simulink model "WSCC01"  (R2024b)
settings: Solver=ode23tb  StartTime=0.0  StopTime=110  MaxStep=1/60  RelTol=1e-4  AbsTol=1e-3  EnableMultiTasking=on
InitFcn:
  | PSSMODEL=1;
  | MB=[1   0.2 30   1.25 40    12 160];
  | 
  | k=[8.3222    2.6014   19.0811    1.9818    3.6841   19.1783  240.6785    2.5684    4.3666   58.7391 7.6960   47.7975    8.7139  296.2463    2.7543    6.5051   47.7755    0.4780   35.4950   18.1866 94.2186]
  | k1=k(1);
  | k2=k(2);
  | k3=k(3);
  | k4=k(4);
  | k5=k(5);
  | k6=k(6);
  | k7=k(7);
  | k8=k(8);
  | k9=k(9);
  | k10=k(10);
  | k11=k(11);
  | k12=k(12);
  | k13=k(13);
  | k14=k(14);
  | k15=k(15);
  | k16=k(16);
  | k17=k(17);
  | k18=k(18);
  | k19=k(19);
  | k20=k(20);
  | k21=k(21);
libraries: spsThreePhaseVIMeasurementLib x12, spsLoadFlowBusLib x9, spsThreePhasePISectionLineLib x6, spsThreePhaseTransformerTwoWindingsLib x3, spsSynchronousMachinepuStandardLib x3, spsExcitationSystemLib x3, spsMultiBandPowerSystemStabilizerLib x3, spsSteamTurbineandGovernorLib x3, spsThreePhaseParallelRLCLoadLib x3, spsThreePhaseDynamicLoadLib x1, spspowerguiLib x1
settings Model: Creator=jp536285  LastModifiedBy=Raju
settings SolverCC: AutoScaleAbsTol=off  AlgebraicLoopSolver=TrustRegion
settings OptimizationCC: LifeSpan=inf
settings DebuggingCC: UnderspecifiedInitializationDetection=Classic  MergeDetectMultiDrivingBlocksExec=none  SolverPrmCheckMsg=warning  StateNameClashWarn=warning  SFUnexpectedBacktrackingDiag=warning  SFNoUnconditionalDefaultTransitionDiag=warning  ArithmeticOperatorsInVariantConditions=warning
settings HardwareCC: ProdBitPerPointer=32  ProdBitPerSizeT=32  ProdBitPerPtrDiffT=32  ProdLargestAtomicFloat=None  ProdIntDivRoundTo=Undefined  ProdEndianess=Unspecified  ProdWordSize=32  ProdHWDeviceType=32-bit Generic
settings ModelReferenceCC: EnableRefExpFcnMdlSchedulingChecks=on  PropagateSignalLabelsOutOfModel=off
settings SFSimCC: SimUseLocalCustomCode=off  CustomCodeUndefinedFunction=UseInterfaceOnly
settings RTWCC: RTWUseLocalCustomCode=off  GPUComputeCapability=3.5
settings CodeAppCC: StateflowObjectComments=on
settings GRTTargetCC: TargetLangStandard=C89/C90 (ANSI)
settings ConfigComp: CovMetricSettings=dw  CovSaveCumulativeToWorkspaceVar=on  CovSaveSingleToWorkspaceVar=on  CovExternalEMLEnable=off
settings SimscapeCC: SimscapeNormalizeSystem=off

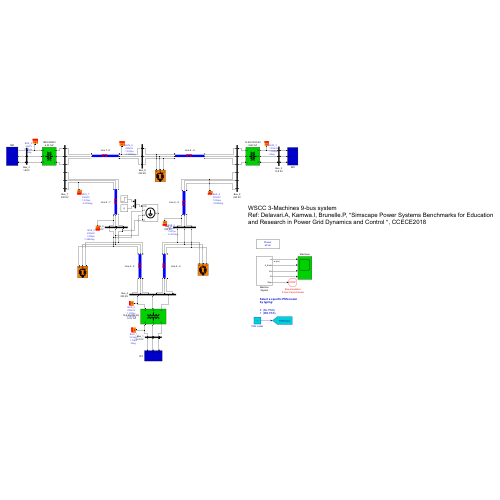
[thumbnail: Simulink's stored preview of the top-level diagram]
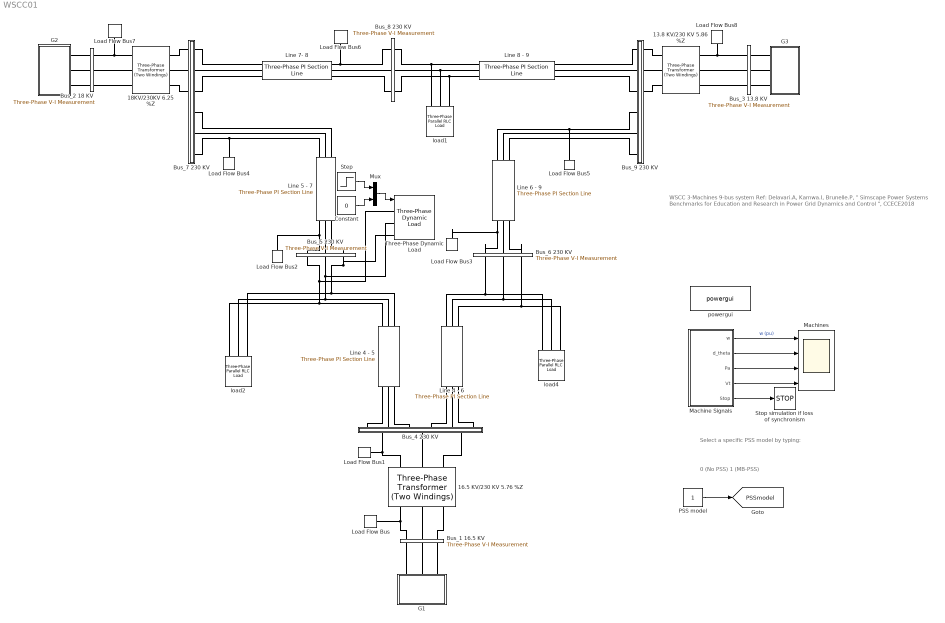
== system WSCC01 ==
  note: WSCC 3-Machines 9-bus system
      | Ref: Delavari.A, Kamwa.I, Brunelle.P, " Simscape Power Systems Benchmarks for Education
      | and Research in Power Grid Dynamics and Control ", CCECE2018
  note: Select a specific PSS model
      | by typing:
  note: 0  (No PSS)
      | 1  (MB-PSS)
  " Line 4 - 6" : spsThreePhasePISectionLineLib/Three-Phase PI Section Line  LConnTagsString=a|b|c  RConnTagsString=A|B|C  Length=100  Frequency=60  Resistances=[ 0.08993 0.224825]  Inductances="[ 1.29e-3  3.22e-3]"  Capacitances="[ 9.5e-9  6.5e-9 ]"  mask(Three-Phase PI Section Line){}
      mask Display:
      | % This is a new mask on top of the base mask.
      | % Use "View base mask" link below to see the base mask.
      | patch([0.0 0.0 1 1 0.0 0.0 ],[0.4 0.7 0.7 0.4 0.4 0.7],[0 0 1]);
      | patch([0.4 0.4 0.42 0.42],[0.4 0.75 0.75 0.4],[1 0 0]);
      | patch([0.38 0.38 0.57 0.57],[0.7 0.75 0.75 0.7],[1 0 0]);
      | patch([0.53 0.53 0.55 0.55],[0.4 0.75 0.75 0.4],[1 0 0]);
  " Line 6 - 9" : spsThreePhasePISectionLineLib/Three-Phase PI Section Line  LConnTagsString=a|b|c  RConnTagsString=A|B|C  Length=100  Frequency=60  Resistances=[ 0.20631 0.5157]  Inductances="[ 2.38e-3  6.09e-3]"  Capacitances=[17.95e-9 10.55e-9]  mask(Three-Phase PI Section Line){}
      mask Display:
      | % This is a new mask on top of the base mask.
      | % Use "View base mask" link below to see the base mask.
      | patch([0.0 0.0 1 1 0.0 0.0 ],[0.4 0.7 0.7 0.4 0.4 0.7],[0 0 1]);
      | patch([0.4 0.4 0.42 0.42],[0.4 0.75 0.75 0.4],[1 0 0]);
      | patch([0.38 0.38 0.57 0.57],[0.7 0.75 0.75 0.7],[1 0 0]);
      | patch([0.53 0.53 0.55 0.55],[0.4 0.75 0.75 0.4],[1 0 0]);
  13.8 KV/230 KV 5.86 %Z : spsThreePhaseTransformerTwoWindingsLib/Three-Phase Transformer (Two Windings)  Winding1Connection=Yg  Winding2Connection=Yg  CoreType=Three single-phase transformers  SetSaturation=off  Hysteresis=off  DataFile='hysteresis'  SetInitialFlux=off  Measurements=None  UNITS=pu  NominalPower=[ 100e6 , 60 ]  Winding1=[ 13.8e3 , 1e-6 , 0 ]  Winding2=[ 230e3 , 1e-6, 0.0586 ]  Rm=500  Lm=500  L0=0.5  Saturation=[ 0,0 ; 0.0024,1.2 ; 1.0,1.52 ]  InitialFluxes=[ 0.8 , -0.8 , 0.7 ]  BreakLoop=off  DiscreteSolver=Trapezoidal iterative  DataType=off  TransfoNumber=1
  "16.5 KV/230 KV 5.76 %Z     " : spsThreePhaseTransformerTwoWindingsLib/Three-Phase Transformer (Two Windings)  Winding1Connection=Yg  Winding2Connection=Yg  CoreType=Three single-phase transformers  SetSaturation=off  Hysteresis=off  DataFile='hysteresis'  SetInitialFlux=off  Measurements=None  UNITS=pu  NominalPower=[ 100e6 , 60 ]  Winding1=[ 16.5e3 , 1e-6, 0 ]  Winding2=[ 230e3 ,1e-6, 0.0576 ]  Rm=500  Lm=500  L0=0.5  Saturation=[ 0,0 ; 0.0024,1.2 ; 1.0,1.52 ]  InitialFluxes=[ 0.8 , -0.8 , 0.7 ]  BreakLoop=off  DiscreteSolver=Trapezoidal iterative  DataType=off  TransfoNumber=1
  18KV/230KV 6.25 %Z : spsThreePhaseTransformerTwoWindingsLib/Three-Phase Transformer (Two Windings)  Winding1Connection=Yg  Winding2Connection=Yg  CoreType=Three single-phase transformers  SetSaturation=off  Hysteresis=off  DataFile='hysteresis'  SetInitialFlux=off  Measurements=None  UNITS=pu  NominalPower=[ 100e6 , 60 ]  Winding1=[ 18e3 , 1e-6 , 0]  Winding2=[ 230e3 , 1e-6, 0.0625 ]  Rm=500  Lm=500  L0=0.5  Saturation=[ 0,0 ; 0.0024,1.2 ; 1.0,1.52 ]  InitialFluxes=[ 0.8 , -0.8 , 0.7 ]  BreakLoop=off  DiscreteSolver=Trapezoidal iterative  DataType=off  TransfoNumber=1
  Bus_1 16.5 KV : spsThreePhaseVIMeasurementLib/Three-Phase V-I Measurement  VoltageMeasurement=phase-to-ground  SetLabelV=on  LabelV=Vabc_1  Vpu=on  VpuLL=off  CurrentMeasurement=yes  SetLabelI=on  LabelI=Iabc_1  Ipu=on  Pbase=100e6  Vbase=16.5e3  OutputType=Complex  PhasorSimulation=on  PSBequivalent=0
  Bus_2 18 KV : spsThreePhaseVIMeasurementLib/Three-Phase V-I Measurement  VoltageMeasurement=phase-to-ground  SetLabelV=on  LabelV=Vabc_2  Vpu=on  VpuLL=off  CurrentMeasurement=yes  SetLabelI=on  LabelI=Iabc_2  Ipu=on  Pbase=100e6  Vbase=18e3  OutputType=Complex  PhasorSimulation=on  PSBequivalent=0
  Bus_3 13.8 KV : spsThreePhaseVIMeasurementLib/Three-Phase V-I Measurement  VoltageMeasurement=phase-to-ground  SetLabelV=on  LabelV=Vabc_3  Vpu=on  VpuLL=off  CurrentMeasurement=yes  SetLabelI=on  LabelI=Iabc_3  Ipu=on  Pbase=100e6  Vbase=13.8e3  OutputType=Complex  PhasorSimulation=on  PSBequivalent=0
  Bus_4 230 KV : Subsystem
  Bus_5 230 KV : spsThreePhaseVIMeasurementLib/Three-Phase V-I Measurement  VoltageMeasurement=phase-to-ground  SetLabelV=on  LabelV=Vabc_5  Vpu=on  VpuLL=off  CurrentMeasurement=yes  SetLabelI=on  LabelI=Iabc_5  Ipu=on  Pbase=100e6  Vbase=230e3  OutputType=Complex  PhasorSimulation=on  PSBequivalent=0
  Bus_6 230 KV : spsThreePhaseVIMeasurementLib/Three-Phase V-I Measurement  VoltageMeasurement=phase-to-phase  SetLabelV=on  LabelV=Vabc_6  Vpu=off  VpuLL=on  CurrentMeasurement=yes  SetLabelI=on  LabelI=Iabc_6  Ipu=on  Pbase=100e6  Vbase=230e3  OutputType=Complex  PhasorSimulation=on  PSBequivalent=0
  Bus_7 230 KV : Subsystem
  Bus_8 230 KV : spsThreePhaseVIMeasurementLib/Three-Phase V-I Measurement  VoltageMeasurement=phase-to-phase  SetLabelV=on  LabelV=Vabc_8  Vpu=off  VpuLL=on  CurrentMeasurement=yes  SetLabelI=on  LabelI=Iabc_8  Ipu=on  Pbase=100e6  Vbase=230e3  OutputType=Complex  PhasorSimulation=on  PSBequivalent=0
  Bus_9 230 KV : Subsystem
  Constant : Constant  Value=0
  G1 : Subsystem
  G2 : Subsystem
  G3 : Subsystem
  "Line 4 - 5 " : spsThreePhasePISectionLineLib/Three-Phase PI Section Line  LConnTagsString=a|b|c  RConnTagsString=A|B|C  Length=100  Frequency=60  Resistances=[ 0.0529 0.13225]  Inductances="[ 1.192e-3  2.38e-3]"  Capacitances="[ 9.5e-9  6.5e-9 ]"  mask(Three-Phase PI Section Line){}
      mask Display:
      | % This is a new mask on top of the base mask.
      | % Use "View base mask" link below to see the base mask.
      | patch([0.0 0.0 1 1 0.0 0.0 ],[0.4 0.7 0.7 0.4 0.4 0.7],[0 0 1]);
      | patch([0.4 0.4 0.42 0.42],[0.4 0.75 0.75 0.4],[1 0 0]);
      | patch([0.38 0.38 0.57 0.57],[0.7 0.75 0.75 0.7],[1 0 0]);
      | patch([0.53 0.53 0.55 0.55],[0.4 0.75 0.75 0.4],[1 0 0]);
  "Line 5 - 7 " : spsThreePhasePISectionLineLib/Three-Phase PI Section Line  LConnTagsString=a|b|c  RConnTagsString=A|B|C  Length=100  Frequency=60  Resistances=[ 0.16928 0.4232]  Inductances="[ 2.259e-3  5.64e-3]"  Capacitances=[15.34e-9 9.025e-9]  mask(Three-Phase PI Section Line){}
      mask Display:
      | % This is a new mask on top of the base mask.
      | % Use "View base mask" link below to see the base mask.
      | patch([0.0 0.0 1 1 0.0 0.0 ],[0.4 0.7 0.7 0.4 0.4 0.7],[0 0 1]);
      | patch([0.4 0.4 0.42 0.42],[0.4 0.75 0.75 0.4],[1 0 0]);
      | patch([0.38 0.38 0.57 0.57],[0.7 0.75 0.75 0.7],[1 0 0]);
      | patch([0.53 0.53 0.55 0.55],[0.4 0.75 0.75 0.4],[1 0 0]);
  Line 7- 8 : spsThreePhasePISectionLineLib/Three-Phase PI Section Line  LConnTagsString=a|b|c  RConnTagsString=A|B|C  Length=100  Frequency=60  Resistances=[0.044965 0.11241]  Inductances="[ 1.01e-3  2.02e-3]"  Capacitances="[ 12.5e-9  6.5e-9 ]"  mask(Three-Phase PI Section Line){}
      mask Display:
      | % This is a new mask on top of the base mask.
      | % Use "View base mask" link below to see the base mask.
      | patch([0.0 0.0 1 1 0.0 0.0 ],[0.4 0.7 0.7 0.4 0.4 0.7],[0 0 1]);
      | patch([0.4 0.4 0.42 0.42],[0.4 0.75 0.75 0.4],[1 0 0]);
      | patch([0.38 0.38 0.57 0.57],[0.7 0.75 0.75 0.7],[1 0 0]);
      | patch([0.53 0.53 0.55 0.55],[0.4 0.75 0.75 0.4],[1 0 0]);
  Line 8 - 9 : spsThreePhasePISectionLineLib/Three-Phase PI Section Line  LConnTagsString=a|b|c  RConnTagsString=A|B|C  Length=100  Frequency=60  Resistances=[ 0.062951 0.15737]  Inductances="[ 1.414e-3  3.53e-3]"  Capacitances=[10.47e-9 6.15e-9]  mask(Three-Phase PI Section Line){}
      mask Display:
      | % This is a new mask on top of the base mask.
      | % Use "View base mask" link below to see the base mask.
      | patch([0.0 0.0 1 1 0.0 0.0 ],[0.4 0.7 0.7 0.4 0.4 0.7],[0 0 1]);
      | patch([0.4 0.4 0.42 0.42],[0.4 0.75 0.75 0.4],[1 0 0]);
      | patch([0.38 0.38 0.57 0.57],[0.7 0.75 0.75 0.7],[1 0 0]);
      | patch([0.53 0.53 0.55 0.55],[0.4 0.75 0.75 0.4],[1 0 0]);
  Load Flow Bus : spsLoadFlowBusLib/Load Flow Bus  LConnTagsString=a  Phases=single  Connectors=on one side  ID=BUS_1  Vbase=16.5e3  Vref=1.04  Vangle=0  VLF=1.04  VLFb=1  VLFc=1  angleLF=0  angleLFb=0  angleLFc=0
      settings: AttributesFormatString=%<ID>\n%<Vbase>V\n%<VLF>pu\n%<angleLF>deg.
  Load Flow Bus1 : spsLoadFlowBusLib/Load Flow Bus  LConnTagsString=a  Phases=single  Connectors=on one side  ID=BUS_4  Vbase=230e3  Vref=1  Vangle=0  VLF=1.032  VLFb=1  VLFc=1  angleLF=-3.967  angleLFb=0  angleLFc=0
      settings: AttributesFormatString=%<ID>\n%<Vbase>V\n%<VLF>pu\n%<angleLF>deg.
  Load Flow Bus2 : spsLoadFlowBusLib/Load Flow Bus  LConnTagsString=a  Phases=single  Connectors=on one side  ID=BUS_5  Vbase=230e3  Vref=1  Vangle=0  VLF=1.006  VLFb=1  VLFc=1  angleLF=-7.488  angleLFb=0  angleLFc=0
      settings: AttributesFormatString=%<ID>\n%<Vbase>V\n%<VLF>pu\n%<angleLF>deg.
  Load Flow Bus3 : spsLoadFlowBusLib/Load Flow Bus  LConnTagsString=a  Phases=single  Connectors=on one side  ID=BUS_6  Vbase=230e3  Vref=1  Vangle=0  VLF=1.021  VLFb=1  VLFc=1  angleLF=-6.451  angleLFb=0  angleLFc=0
      settings: AttributesFormatString=%<ID>\n%<Vbase>V\n%<VLF>pu\n%<angleLF>deg.
  Load Flow Bus4 : spsLoadFlowBusLib/Load Flow Bus  LConnTagsString=a  Phases=single  Connectors=on one side  ID=BUS_7  Vbase=230e3  Vref=1  Vangle=0  VLF=1.032  VLFb=1  VLFc=1  angleLF=-3.393  angleLFb=0  angleLFc=0
      settings: AttributesFormatString=%<ID>\n%<Vbase>V\n%<VLF>pu\n%<angleLF>deg.
  Load Flow Bus5 : spsLoadFlowBusLib/Load Flow Bus  LConnTagsString=a  Phases=single  Connectors=on one side  ID=BUS_9  Vbase=230e3  Vref=1  Vangle=0  VLF=1.036  VLFb=1  VLFc=1  angleLF=-2.808  angleLFb=0  angleLFc=0
      settings: AttributesFormatString=%<ID>\n%<Vbase>V\n%<VLF>pu\n%<angleLF>deg.
  Load Flow Bus6 : spsLoadFlowBusLib/Load Flow Bus  LConnTagsString=a  Phases=single  Connectors=on one side  ID=BUS_8  Vbase=230e3  Vref=1  Vangle=0  VLF=1.023  VLFb=1  VLFc=1  angleLF=-5.389  angleLFb=0  angleLFc=0
      settings: AttributesFormatString=%<ID>\n%<Vbase>V\n%<VLF>pu\n%<angleLF>deg.
  Load Flow Bus7 : spsLoadFlowBusLib/Load Flow Bus  LConnTagsString=a  Phases=single  Connectors=on one side  ID=BUS_2  Vbase=18e3  Vref=1.025  Vangle=0  VLF=1.025  VLFb=1  VLFc=1  angleLF=0  angleLFb=0  angleLFc=0
      settings: AttributesFormatString=%<ID>\n%<Vbase>V\n%<VLF>pu\n%<angleLF>deg.
  Load Flow Bus8 : spsLoadFlowBusLib/Load Flow Bus  LConnTagsString=a  Phases=single  Connectors=on one side  ID=BUS_3  Vbase=13.8e3  Vref=1.025  Vangle=0  VLF=1.025  VLFb=1  VLFc=1  angleLF=0  angleLFb=0  angleLFc=0
      settings: AttributesFormatString=%<ID>\n%<Vbase>V\n%<VLF>pu\n%<angleLF>deg.
  Machine Signals : Subsystem
  Machines : Scope  NumInputPorts=4
  Mux : Mux  Inputs=2
  PSS model : Constant
  Step : Step  Time=50  After=30e6  SampleTime=0
  Stop simulation if loss of synchronism : Stop
  Three-Phase Dynamic Load : spsThreePhaseDynamicLoadLib/Three-Phase Dynamic Load  NominalVoltage=[ 230e3 60 ]  ActiveReactivePowers=[0 0]  PositiveSequence=[1.00595 -7.48802]  ExternalControl=on  NpNq=[1.3 2]  TimeConstants="[0  0  0  0]"  MinimumVoltage=0.7  Tfilter=1e-4  LoadFlowParameters=[4,0,0,0,0]
      settings: LibrarySourceBlock=|
      | sps_lib/Passives/Three-Phase
      | Dynamic Load
  load1 : spsThreePhaseParallelRLCLoadLib/Three-Phase Parallel RLC Load  LConnTagsString=A|B|C  Configuration=Y (grounded)  NominalVoltage=(230000)*1.02319  Vabc=[1e3 1e3 1e3]  Vabcp=[1e3 1e3 1e3]  NominalFrequency=60  UnbalancedPower=off  ActivePower=100000000  InductivePower=35000000  CapacitivePower=0  Pabc=[10e3 9e3 11e3]  QLabc=[100 90 110]  QCabc=[100 90 110]  Pabcp=[10e3 9e3 11e3]  QLabcp=[100 90 110]  QCabcp=[100 90 110]  Measurements=None  LoadType=constant PQ
  load2 : spsThreePhaseParallelRLCLoadLib/Three-Phase Parallel RLC Load  LConnTagsString=A|B|C  Configuration=Y (grounded)  NominalVoltage=(230000)*1.00595  Vabc=[1e3 1e3 1e3]  Vabcp=[1e3 1e3 1e3]  NominalFrequency=60  UnbalancedPower=off  ActivePower=125000000  InductivePower=50000000  CapacitivePower=0  Pabc=[10e3 9e3 11e3]  QLabc=[100 90 110]  QCabc=[100 90 110]  Pabcp=[10e3 9e3 11e3]  QLabcp=[100 90 110]  QCabcp=[100 90 110]  Measurements=None  LoadType=constant PQ
  load4 : spsThreePhaseParallelRLCLoadLib/Three-Phase Parallel RLC Load  LConnTagsString=A|B|C  Configuration=Y (grounded)  NominalVoltage=(230000)*1.02056  Vabc=[1e3 1e3 1e3]  Vabcp=[1e3 1e3 1e3]  NominalFrequency=60  UnbalancedPower=off  ActivePower=90000000  InductivePower=30000000  CapacitivePower=0  Pabc=[10e3 9e3 11e3]  QLabc=[100 90 110]  QCabc=[100 90 110]  Pabcp=[10e3 9e3 11e3]  QLabcp=[100 90 110]  QCabcp=[100 90 110]  Measurements=None  LoadType=constant PQ
  powergui : spspowerguiLib/powergui  Priority=1  SimulationMode=Phasor  SampleTime=50e-6  frequency=60  Iterations=50  frequencyindice=60  Pbase=10e7  ErrMax=1e-05  UnitsV=kV  UnitsW=MW  buscounter=0  FunctionMessages=off  echomessages=off  EnableUseOfTLC=off  CurrentSourceSwitches=off  DisableSnubberDevices=off  DisableRonSwitches=off  DisableVfSwitches=off  DisplayEquations=off  AutomaticDiscreteSolvers=off  SolverType=Tustin  Interpol=off  ExternalGateDelay=off  methode=off  Ts=0  x0status=blocks  SPID=off  SwTol=0  HookPort=off  NonlinearTolerance=1e-4  nMaxIteration=100  ContinueOnMaxIteration=off  RestoreLinks=warning  ResistiveCurrentMeasurement=off  Frange=[0:2:500]  Ylog=off  Xlog=on  ShowGrid=off  save=off  variable=ZData  structure=0  ZoomFFT=off  StartTime=0.0  cycles=1  DisplayStyle=1  fundamental=60  FreqAxis=off  MaxFrequency=1000  frequencyindicesteady=1  RmsSteady=1  display=off
  tag scope: PSSmodel=global
  wires:
  Machine Signals/1(w) -> Machines/1  "w (pu)"
  Machine Signals/2(d_theta) -> Machines/2
  Machine Signals/3(Pa) -> Machines/3
  Machine Signals/4(Vt) -> Machines/4
  PSS model/1 -> [PSSmodel]
  Machine Signals/5(Stop) -> Stop simulation if loss of synchronism/1
  Step/1 -> Mux/1
  Constant/1 -> Mux/2
  Mux/1 -> Three-Phase Dynamic Load/1
  connections:
  G2/LConn2 -- Bus_2 18 KV/LConn2
  18KV/230KV 6.25 %Z/LConn2 -- Bus_2 18 KV/RConn2
  18KV/230KV 6.25 %Z/RConn2 -- Bus_7 230 KV/LConn2
  Bus_2 18 KV/RConn1 -- 18KV/230KV 6.25 %Z/LConn1 -- Load Flow Bus7/LConn1
  Bus_2 18 KV/RConn3 -- 18KV/230KV 6.25 %Z/LConn3
  Bus_7 230 KV/LConn1 -- 18KV/230KV 6.25 %Z/RConn1
  18KV/230KV 6.25 %Z/RConn3 -- Bus_7 230 KV/LConn3
  Load Flow Bus8/LConn1 -- 13.8 KV/230 KV 5.86 %Z/LConn1 -- Bus_3 13.8 KV/LConn1
  13.8 KV/230 KV 5.86 %Z/LConn2 -- Bus_3 13.8 KV/LConn2
  13.8 KV/230 KV 5.86 %Z/LConn3 -- Bus_3 13.8 KV/LConn3
  Bus_1 16.5 KV/LConn1 -- Load Flow Bus/LConn1 -- "16.5 KV/230 KV 5.76 %Z     "/LConn1
  Bus_1 16.5 KV/LConn3 -- "16.5 KV/230 KV 5.76 %Z     "/LConn3
  Bus_1 16.5 KV/LConn2 -- "16.5 KV/230 KV 5.76 %Z     "/LConn2
  13.8 KV/230 KV 5.86 %Z/RConn1 -- Bus_9 230 KV/RConn1
  13.8 KV/230 KV 5.86 %Z/RConn2 -- Bus_9 230 KV/RConn2
  13.8 KV/230 KV 5.86 %Z/RConn3 -- Bus_9 230 KV/RConn3
  Bus_4 230 KV/LConn1 -- "16.5 KV/230 KV 5.76 %Z     "/RConn1 -- Load Flow Bus1/LConn1
  Bus_4 230 KV/LConn2 -- "16.5 KV/230 KV 5.76 %Z     "/RConn2
  Line 8 - 9/LConn1 -- load1/LConn1 -- Bus_8 230 KV/LConn1
  Bus_8 230 KV/LConn2 -- load1/LConn2 -- Line 8 - 9/LConn2
  Line 8 - 9/LConn3 -- load1/LConn3 -- Bus_8 230 KV/LConn3
  "16.5 KV/230 KV 5.76 %Z     "/RConn3 -- Bus_4 230 KV/LConn3
  "Line 4 - 5 "/LConn1 -- Three-Phase Dynamic Load/LConn1 -- Bus_5 230 KV/RConn1 -- load2/LConn1
  "Line 4 - 5 "/LConn2 -- load2/LConn2 -- Three-Phase Dynamic Load/LConn2 -- Bus_5 230 KV/RConn2
  "Line 4 - 5 "/LConn3 -- Three-Phase Dynamic Load/LConn3 -- Bus_5 230 KV/RConn3 -- load2/LConn3
  " Line 4 - 6"/LConn1 -- load4/LConn1 -- Bus_6 230 KV/RConn1
  " Line 4 - 6"/LConn2 -- load4/LConn2 -- Bus_6 230 KV/RConn2
  " Line 4 - 6"/LConn3 -- load4/LConn3 -- Bus_6 230 KV/RConn3
  Line 7- 8/LConn1 -- Bus_7 230 KV/RConn1
  Line 7- 8/LConn2 -- Bus_7 230 KV/RConn2
  Bus_7 230 KV/RConn3 -- Line 7- 8/LConn3
  Bus_8 230 KV/RConn1 -- Load Flow Bus6/LConn1 -- Line 7- 8/RConn1
  Line 7- 8/RConn2 -- Bus_8 230 KV/RConn2
  Line 7- 8/RConn3 -- Bus_8 230 KV/RConn3
  Line 8 - 9/RConn2 -- Bus_9 230 KV/LConn2
  Line 8 - 9/RConn1 -- Bus_9 230 KV/LConn1
  Line 8 - 9/RConn3 -- Bus_9 230 KV/LConn3
  "Line 5 - 7 "/RConn1 -- Bus_5 230 KV/LConn1 -- Load Flow Bus2/LConn1
  "Line 5 - 7 "/RConn2 -- Bus_5 230 KV/LConn2
  "Line 5 - 7 "/RConn3 -- Bus_5 230 KV/LConn3
  "Line 5 - 7 "/LConn1 -- Load Flow Bus4/LConn1 -- Bus_7 230 KV/RConn6
  "Line 5 - 7 "/LConn2 -- Bus_7 230 KV/RConn5
  "Line 5 - 7 "/LConn3 -- Bus_7 230 KV/RConn4
  " Line 6 - 9"/RConn1 -- Load Flow Bus5/LConn1 -- Bus_9 230 KV/LConn4
  Bus_9 230 KV/LConn5 -- " Line 6 - 9"/RConn2
  Bus_6 230 KV/LConn1 -- Load Flow Bus3/LConn1 -- " Line 6 - 9"/LConn1
  Bus_6 230 KV/LConn2 -- " Line 6 - 9"/LConn2
  Bus_6 230 KV/LConn3 -- " Line 6 - 9"/LConn3
  " Line 6 - 9"/RConn3 -- Bus_9 230 KV/LConn6
  "Line 4 - 5 "/RConn2 -- Bus_4 230 KV/RConn2
  "Line 4 - 5 "/RConn1 -- Bus_4 230 KV/RConn1
  "Line 4 - 5 "/RConn3 -- Bus_4 230 KV/RConn3
  " Line 4 - 6"/RConn2 -- Bus_4 230 KV/RConn5
  " Line 4 - 6"/RConn1 -- Bus_4 230 KV/RConn4
  " Line 4 - 6"/RConn3 -- Bus_4 230 KV/RConn6
  G3/LConn1 -- Bus_3 13.8 KV/RConn1
  G3/LConn2 -- Bus_3 13.8 KV/RConn2
  G3/LConn3 -- Bus_3 13.8 KV/RConn3
  G2/LConn3 -- Bus_2 18 KV/LConn3
  G2/LConn1 -- Bus_2 18 KV/LConn1
  G1/LConn1 -- Bus_1 16.5 KV/RConn1
  G1/LConn2 -- Bus_1 16.5 KV/RConn2
  G1/LConn3 -- Bus_1 16.5 KV/RConn3

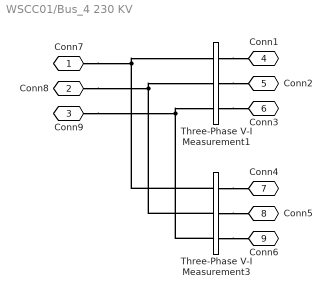
== system WSCC01/Bus_4 230 KV ==
  Three-Phase V-I Measurement1 : spsThreePhaseVIMeasurementLib/Three-Phase V-I Measurement  VoltageMeasurement=phase-to-ground  SetLabelV=on  LabelV=Vabc_45  Vpu=on  VpuLL=off  CurrentMeasurement=yes  SetLabelI=on  LabelI=Iabc_45  Ipu=on  Pbase=100e6  Vbase=230e3  OutputType=Complex  PhasorSimulation=on  PSBequivalent=0
  Three-Phase V-I Measurement3 : spsThreePhaseVIMeasurementLib/Three-Phase V-I Measurement  VoltageMeasurement=phase-to-ground  SetLabelV=on  LabelV=Vabc_46  Vpu=on  VpuLL=off  CurrentMeasurement=yes  SetLabelI=on  LabelI=Iabc_46  Ipu=on  Pbase=100e6  Vbase=230e3  OutputType=Complex  PhasorSimulation=on  PSBequivalent=0
  Conn7 : PMIOPort  Side=Left
  Conn8 : PMIOPort  Port=2  Side=Left
  Conn9 : PMIOPort  Port=3  Side=Left
  Conn1 : PMIOPort  Port=4  Side=Right
  Conn2 : PMIOPort  Port=5  Side=Right
  Conn3 : PMIOPort  Port=6  Side=Right
  Conn4 : PMIOPort  Port=7  Side=Right
  Conn5 : PMIOPort  Port=8  Side=Right
  Conn6 : PMIOPort  Port=9  Side=Right
  connections:
  Three-Phase V-I Measurement3/LConn3 -- Conn9/RConn1 -- Three-Phase V-I Measurement1/LConn3
  Three-Phase V-I Measurement3/LConn2 -- Conn8/RConn1 -- Three-Phase V-I Measurement1/LConn2
  Three-Phase V-I Measurement3/LConn1 -- Conn7/RConn1 -- Three-Phase V-I Measurement1/LConn1
  Three-Phase V-I Measurement3/RConn3 -- Conn6/RConn1
  Three-Phase V-I Measurement1/RConn3 -- Conn3/RConn1
  Three-Phase V-I Measurement1/RConn1 -- Conn1/RConn1
  Three-Phase V-I Measurement1/RConn2 -- Conn2/RConn1
  Three-Phase V-I Measurement3/RConn1 -- Conn4/RConn1
  Three-Phase V-I Measurement3/RConn2 -- Conn5/RConn1

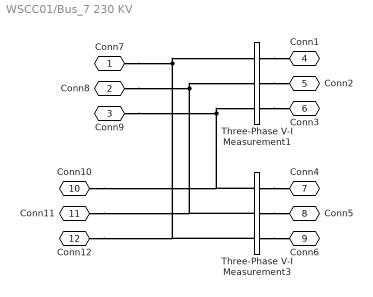
== system WSCC01/Bus_7 230 KV ==
  Three-Phase V-I Measurement1 : spsThreePhaseVIMeasurementLib/Three-Phase V-I Measurement  VoltageMeasurement=phase-to-ground  SetLabelV=on  LabelV=Vabc_7  Vpu=on  VpuLL=off  CurrentMeasurement=yes  SetLabelI=on  LabelI=Iabc_7  Ipu=on  Pbase=100e6  Vbase=230e3  OutputType=Complex  PhasorSimulation=on  PSBequivalent=0
  Three-Phase V-I Measurement3 : spsThreePhaseVIMeasurementLib/Three-Phase V-I Measurement  VoltageMeasurement=phase-to-ground  SetLabelV=on  LabelV=Vab  Vpu=on  VpuLL=off  CurrentMeasurement=yes  SetLabelI=on  LabelI=Iab  Ipu=on  Pbase=100e6  Vbase=230e3  OutputType=Complex  PhasorSimulation=on  PSBequivalent=0
  Conn7 : PMIOPort  Side=Left
  Conn8 : PMIOPort  Port=2  Side=Left
  Conn9 : PMIOPort  Port=3  Side=Left
  Conn1 : PMIOPort  Port=4  Side=Right
  Conn2 : PMIOPort  Port=5  Side=Right
  Conn3 : PMIOPort  Port=6  Side=Right
  Conn4 : PMIOPort  Port=7  Side=Right
  Conn5 : PMIOPort  Port=8  Side=Right
  Conn6 : PMIOPort  Port=9  Side=Right
  Conn10 : PMIOPort  Port=10  Side=Left
  Conn11 : PMIOPort  Port=11  Side=Left
  Conn12 : PMIOPort  Port=12  Side=Left
  connections:
  Three-Phase V-I Measurement3/RConn2 -- Conn5/RConn1
  Three-Phase V-I Measurement3/RConn1 -- Conn4/RConn1
  Three-Phase V-I Measurement1/RConn2 -- Conn2/RConn1
  Three-Phase V-I Measurement1/RConn1 -- Conn1/RConn1
  Three-Phase V-I Measurement1/RConn3 -- Conn3/RConn1
  Three-Phase V-I Measurement3/RConn3 -- Conn6/RConn1
  Conn7/RConn1 -- Three-Phase V-I Measurement3/LConn3 -- Conn12/RConn1 -- Three-Phase V-I Measurement1/LConn1
  Conn8/RConn1 -- Three-Phase V-I Measurement3/LConn2 -- Conn11/RConn1 -- Three-Phase V-I Measurement1/LConn2
  Conn9/RConn1 -- Conn10/RConn1 -- Three-Phase V-I Measurement3/LConn1 -- Three-Phase V-I Measurement1/LConn3

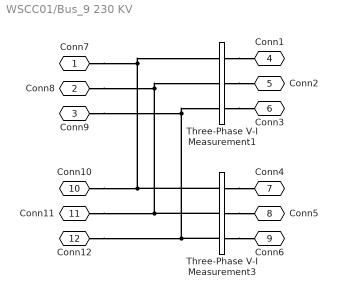
== system WSCC01/Bus_9 230 KV ==
  Three-Phase V-I Measurement1 : spsThreePhaseVIMeasurementLib/Three-Phase V-I Measurement  VoltageMeasurement=phase-to-ground  SetLabelV=on  LabelV=Vabc_9  Vpu=on  VpuLL=off  CurrentMeasurement=yes  SetLabelI=on  LabelI=Iabc_9  Ipu=on  Pbase=100e6  Vbase=230e3  OutputType=Complex  PhasorSimulation=on  PSBequivalent=0
  Three-Phase V-I Measurement3 : spsThreePhaseVIMeasurementLib/Three-Phase V-I Measurement  VoltageMeasurement=phase-to-ground  SetLabelV=on  LabelV=Vabc  Vpu=on  VpuLL=off  CurrentMeasurement=yes  SetLabelI=on  LabelI=Iabc  Ipu=on  Pbase=100e6  Vbase=230e3  OutputType=Complex  PhasorSimulation=on  PSBequivalent=0
  Conn7 : PMIOPort  Side=Left
  Conn8 : PMIOPort  Port=2  Side=Left
  Conn9 : PMIOPort  Port=3  Side=Left
  Conn1 : PMIOPort  Port=4  Side=Right
  Conn2 : PMIOPort  Port=5  Side=Right
  Conn3 : PMIOPort  Port=6  Side=Right
  Conn4 : PMIOPort  Port=7  Side=Right
  Conn5 : PMIOPort  Port=8  Side=Right
  Conn6 : PMIOPort  Port=9  Side=Right
  Conn10 : PMIOPort  Port=10  Side=Left
  Conn11 : PMIOPort  Port=11  Side=Left
  Conn12 : PMIOPort  Port=12  Side=Left
  connections:
  Conn12/RConn1 -- Three-Phase V-I Measurement3/LConn3 -- Conn9/RConn1 -- Three-Phase V-I Measurement1/LConn3
  Conn11/RConn1 -- Three-Phase V-I Measurement3/LConn2 -- Conn8/RConn1 -- Three-Phase V-I Measurement1/LConn2
  Conn10/RConn1 -- Three-Phase V-I Measurement3/LConn1 -- Conn7/RConn1 -- Three-Phase V-I Measurement1/LConn1
  Three-Phase V-I Measurement3/RConn3 -- Conn6/RConn1
  Three-Phase V-I Measurement1/RConn3 -- Conn3/RConn1
  Three-Phase V-I Measurement1/RConn1 -- Conn1/RConn1
  Three-Phase V-I Measurement1/RConn2 -- Conn2/RConn1
  Three-Phase V-I Measurement3/RConn1 -- Conn4/RConn1
  Three-Phase V-I Measurement3/RConn2 -- Conn5/RConn1

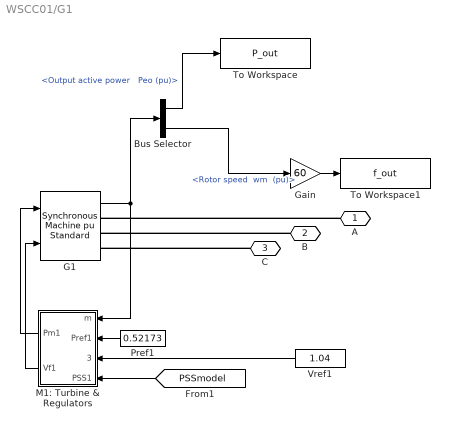
== system WSCC01/G1 ==
  Bus Selector : BusSelector  OutputSignals="Output active power   Peo (pu),Mechanical.Rotor speed  wm  (pu)"
  G1 : spsSynchronousMachinepuStandardLib/Synchronous Machine pu Standard  PresetModel=No  MechanicalLoad=Mechanical power Pm  ShowDetailedParameters=on  RotorType=Round  Units=per unit standard parameters  MeasurementBus=off  NominalParameters="[247.5e6  16500   60 ]"  Reactances1=[1.146 0.2998 0.25 0.969 0.45 0.25 0.025]  Reactances2=[ 1.305, 0.296, 0.252, 0.474, 0.243, 0.18 ]  dAxisTimeConstants=Open-circuit  qAxisTimeConstants=Open-circuit  TimeConstants1=[]  TimeConstants2=[8.96 0.05 0.31 0.05]  TimeConstants3=[]  TimeConstants4=[]  TimeConstants5=[ 1.01, 0.053, 0.1 ]  TimeConstants6=[]  TimeConstants7=[]  TimeConstants8=[]  StatorResistance=0.0025  Mechanical="[ 23.64  0  4]"  PolePairs=4  InitialConditions=[0 -66.3996 0.506988 0.506988 0.506988 -8.3077 -128.308 111.692 1.26119]  SetSaturation=off  Saturation=[0.6404,0.7127,0.8441,0.9214,0.9956,1.082,1.19,1.316,1.457;0.7,0.7698,0.8872,0.9466,0.9969,1.046,1.1,1.151,1.201]  LoadFlowParameters=[2 128000000 0 0 0]  TsPowergui=0  TsBlock=-1  IterativeModel=Forward Euler  IterativeDiscreteModel=Trapezoidal non iterative  BusType=swing  Pref=NaN  Qref=0  Qmin=-Inf  Qmax=Inf  PLF=0  QLF=0
  Gain : Gain  Gain=60
  M1: Turbine & Regulators : Subsystem
  Pref1 : Constant  Value=0.52173
  To Workspace : ToWorkspace  VariableName=P_out  SaveFormat=Timeseries  SampleTime=-1
  To Workspace1 : ToWorkspace  VariableName=f_out  SaveFormat=Timeseries  SampleTime=-1
  Vref1 : Constant  Value=1.04
  A : PMIOPort  Side=Left
  B : PMIOPort  Port=2  Side=Left
  C : PMIOPort  Port=3  Side=Left
  wires:
  Pref1/1 -> M1: Turbine & Regulators/2(Pref1)
  [PSSmodel] -> M1: Turbine & Regulators/4(PSS1)
  M1: Turbine & Regulators/1(Pm1) -> G1/1
  M1: Turbine & Regulators/2(Vf1) -> G1/2
  G1/1 -> Bus Selector/1, M1: Turbine & Regulators/1(m)
  Vref1/1 -> M1: Turbine & Regulators/3(Vref1)
  Bus Selector/1 -> To Workspace/1  "<Output active power   Peo (pu)>"
  Bus Selector/2 -> Gain/1  "<Rotor speed  wm  (pu)>"
  Gain/1 -> To Workspace1/1
  connections:
  A/RConn1 -- G1/RConn1
  B/RConn1 -- G1/RConn2
  C/RConn1 -- G1/RConn3

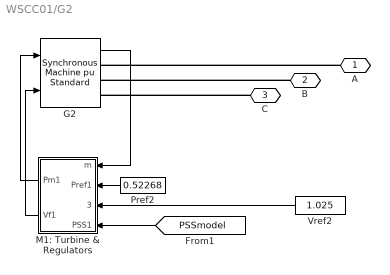
== system WSCC01/G2 ==
  G2 : spsSynchronousMachinepuStandardLib/Synchronous Machine pu Standard  PresetModel=No  MechanicalLoad=Mechanical power Pm  ShowDetailedParameters=on  RotorType=Round  Units=per unit standard parameters  MeasurementBus=off  NominalParameters="[192e6  18000   60 ]"  Reactances1=[0.8958 0.2998 0.25 0.8645 0.45 0.25 0.025]  Reactances2=[ 1.305, 0.296, 0.252, 0.474, 0.243, 0.18 ]  dAxisTimeConstants=Open-circuit  qAxisTimeConstants=Open-circuit  TimeConstants1=[]  TimeConstants2=[6.0 0.05 0.535 0.05]  TimeConstants3=[]  TimeConstants4=[]  TimeConstants5=[ 1.01, 0.053, 0.1 ]  TimeConstants6=[]  TimeConstants7=[]  TimeConstants8=[]  StatorResistance=0.0025  Mechanical="[ 6.4  0  4]"  PolePairs=4  InitialConditions=[0 -66.0422 0.511446 0.511446 0.511446 4.40329 -115.597 124.403 1.09124]  SetSaturation=off  Saturation=[0.6404,0.7127,0.8441,0.9214,0.9956,1.082,1.19,1.316,1.457;0.7,0.7698,0.8872,0.9466,0.9969,1.046,1.1,1.151,1.201]  LoadFlowParameters=[1 1000000000 0 0 0]  TsPowergui=0  TsBlock=-1  IterativeModel=Forward Euler  IterativeDiscreteModel=Trapezoidal non iterative  BusType=PV  Pref=163e6  Qref=0  Qmin=-Inf  Qmax=Inf  PLF=0  QLF=0
  M1: Turbine & Regulators : Subsystem
  Pref2 : Constant  Value=0.52268
  Vref2 : Constant  Value=1.025
  A : PMIOPort  Side=Left
  B : PMIOPort  Port=2  Side=Left
  C : PMIOPort  Port=3  Side=Left
  wires:
  Pref2/1 -> M1: Turbine & Regulators/2(Pref1)
  [PSSmodel] -> M1: Turbine & Regulators/4(PSS1)
  M1: Turbine & Regulators/1(Pm1) -> G2/1
  M1: Turbine & Regulators/2(Vf1) -> G2/2
  G2/1 -> M1: Turbine & Regulators/1(m)
  Vref2/1 -> M1: Turbine & Regulators/3(Vref1)
  connections:
  A/RConn1 -- G2/RConn1
  B/RConn1 -- G2/RConn2
  C/RConn1 -- G2/RConn3

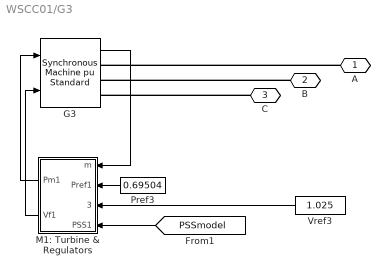
== system WSCC01/G3 ==
  G3 : spsSynchronousMachinepuStandardLib/Synchronous Machine pu Standard  PresetModel=No  MechanicalLoad=Mechanical power Pm  ShowDetailedParameters=on  RotorType=Round  Units=per unit standard parameters  MeasurementBus=off  NominalParameters="[128e6  13800   60 ]"  Reactances1=[1.3125 0.2998 0.25 1.2578 0.45 0.25 0.025]  Reactances2=[ 1.305, 0.296, 0.252, 0.474, 0.243, 0.18 ]  dAxisTimeConstants=Open-circuit  qAxisTimeConstants=Open-circuit  TimeConstants1=[]  TimeConstants2=[5.89 0.05 0.6 0.05]  TimeConstants3=[]  TimeConstants4=[]  TimeConstants5=[ 1.01, 0.053, 0.1 ]  TimeConstants6=[]  TimeConstants7=[]  TimeConstants8=[]  StatorResistance=0.0025  Mechanical="[ 3.01  0  4]"  PolePairs=4  InitialConditions=[0 -45.6071 0.689224 0.689224 0.689224 10.3139 -109.686 130.314 1.24073]  SetSaturation=off  Saturation=[0.6404,0.7127,0.8441,0.9214,0.9956,1.082,1.19,1.316,1.457;0.7,0.7698,0.8872,0.9466,0.9969,1.046,1.1,1.151,1.201]  LoadFlowParameters=[1 1000000000 0 0 0]  TsPowergui=0  TsBlock=-1  IterativeModel=Forward Euler  IterativeDiscreteModel=Trapezoidal non iterative  BusType=PV  Pref=85e6  Qref=0  Qmin=-Inf  Qmax=Inf  PLF=0  QLF=0
  M1: Turbine & Regulators : Subsystem
  Pref3 : Constant  Value=0.69504
  Vref3 : Constant  Value=1.025
  A : PMIOPort  Side=Left
  B : PMIOPort  Port=2  Side=Left
  C : PMIOPort  Port=3  Side=Left
  wires:
  Vref3/1 -> M1: Turbine & Regulators/3(Vref1)
  G3/1 -> M1: Turbine & Regulators/1(m)
  M1: Turbine & Regulators/2(Vf1) -> G3/2
  M1: Turbine & Regulators/1(Pm1) -> G3/1
  [PSSmodel] -> M1: Turbine & Regulators/4(PSS1)
  Pref3/1 -> M1: Turbine & Regulators/2(Pref1)
  connections:
  C/RConn1 -- G3/RConn3
  B/RConn1 -- G3/RConn2
  A/RConn1 -- G3/RConn1

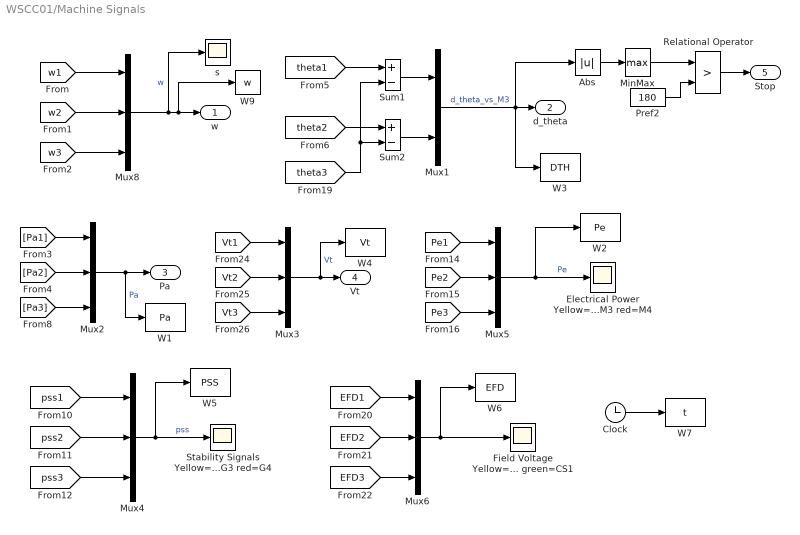
== system WSCC01/Machine Signals ==
  Abs : Abs
  Clock : Clock
  "Electrical Power Yellow=M1 mag=M2 cyan=M3 red=M4 " : Scope
  Field Voltage Yellow=G1 mag=G2 cyan=G3 red=G4 green=CS1 : Scope
  MinMax : MinMax  Function=max  InputSameDT=on  SaturateOnIntegerOverflow=on
  Mux1 : Mux  Inputs=2
  Mux{2..6,8} (6 alike) : Mux  Inputs=3
  Pref2 : Constant  Value=180
  Relational Operator : RelationalOperator  Operator=>
  "Stability Signals Yellow=G1 mag=G2 cyan=G3 red=G4 " : Scope
  Sum1 : Sum  Inputs=+-  InputSameDT=on  SaturateOnIntegerOverflow=on  OutDataTypeStr=Inherit: Same as first input
  Sum2 : Sum  Inputs=+-  InputSameDT=on  SaturateOnIntegerOverflow=on  OutDataTypeStr=Inherit: Same as first input
  W1 : ToWorkspace  VariableName=Pa  SaveFormat=Timeseries  SampleTime=1/60
  W2 : ToWorkspace  VariableName=Pe  SaveFormat=Timeseries  SampleTime=1/60
  W3 : ToWorkspace  VariableName=DTH  SaveFormat=Timeseries  SampleTime=1/60
  W4 : ToWorkspace  VariableName=Vt  SaveFormat=Timeseries  SampleTime=1/60
  W5 : ToWorkspace  VariableName=PSS  SaveFormat=Timeseries  SampleTime=1/60
  W6 : ToWorkspace  VariableName=EFD  SaveFormat=Timeseries  SampleTime=1/60
  W7 : ToWorkspace  VariableName=t  SaveFormat=Timeseries  SampleTime=1/60
  W9 : ToWorkspace  VariableName=w  SaveFormat=Timeseries  SampleTime=1/60
  s : Scope
  w : Outport
  d_theta : Outport  Port=2
  Pa : Outport  Port=3
  Vt : Outport  Port=4
  Stop : Outport  Port=5
  wires:
  Mux8/1 -> s/1, W9/1, w/1  "w"
  [w1] -> Mux8/1
  [w2] -> Mux8/2
  [w3] -> Mux8/3
  Mux1/1 -> d_theta/1, Abs/1, W3/1  "d_theta_vs_M3"
  Abs/1 -> MinMax/1
  Pref2/1 -> Relational Operator/2
  MinMax/1 -> Relational Operator/1
  [Pa1] -> Mux2/1
  Mux4/1 -> "Stability Signals Yellow=G1 mag=G2 cyan=G3 red=G4 "/1, W5/1  "pss"
  [pss1] -> Mux4/1
  [pss2] -> Mux4/2
  [pss3] -> Mux4/3
  [EFD1] -> Mux6/1
  [EFD2] -> Mux6/2
  [EFD3] -> Mux6/3
  Mux6/1 -> Field Voltage Yellow=G1 mag=G2 cyan=G3 red=G4 green=CS1/1, W6/1
  Relational Operator/1 -> Stop/1
  Mux2/1 -> Pa/1, W1/1  "Pa"
  [theta1] -> Sum1/1
  Sum1/1 -> Mux1/1
  [theta2] -> Sum2/1
  [theta3] -> Sum1/2, Sum2/2
  Sum2/1 -> Mux1/2
  [Pa2] -> Mux2/2
  [Pa3] -> Mux2/3
  [Vt1] -> Mux3/1
  [Vt2] -> Mux3/2
  [Vt3] -> Mux3/3
  Mux3/1 -> Vt/1, W4/1  "Vt"
  [Pe1] -> Mux5/1
  [Pe2] -> Mux5/2
  [Pe3] -> Mux5/3
  Mux5/1 -> "Electrical Power Yellow=M1 mag=M2 cyan=M3 red=M4 "/1, W2/1  "Pe"
  Clock/1 -> W7/1

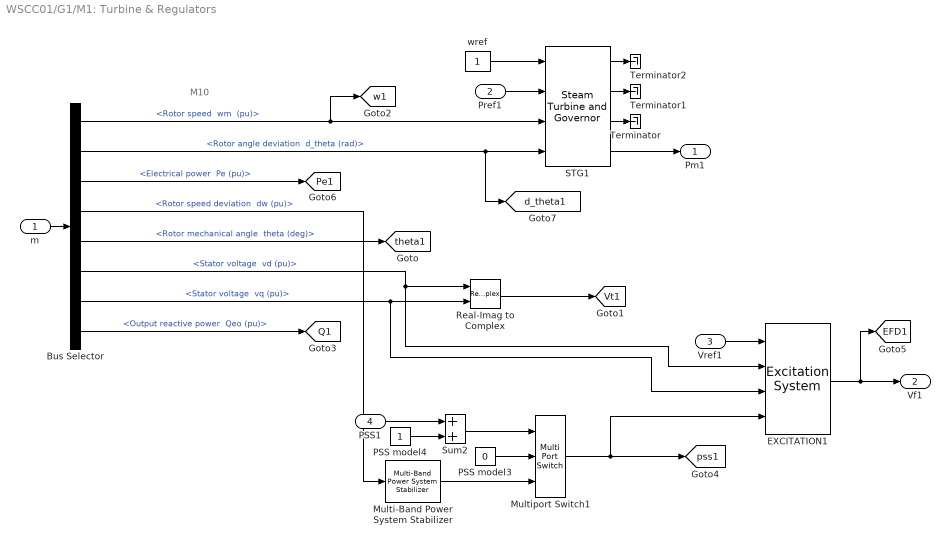
== system WSCC01/G1/M1: Turbine & Regulators ==
  note: M10
  m : Inport
  Pref1 : Inport  Port=2
  Vref1 : Inport  Port=3
  PSS1 : Inport  Port=4
  Bus Selector : BusSelector  OutputSignals="Mechanical.Rotor speed  wm  (pu),Mechanical.Rotor angle deviation  d_theta (rad),Mechanical.Electrical power  Pe (pu),Mechanical.Rotor speed deviation  dw (pu),Mechanical.Rotor mechanical angle  theta (deg),dq0 components.Stator voltage  vd (pu),dq0 components.Stator voltage  vq (pu),Output reactive power  Qeo (pu)"
  EXCITATION1 : spsExcitationSystemLib/Excitation System  tr=0.01  reg=[20 0.2 ]  exc=[ 1, 0.314 ]  tgr=[10 1]  damp=[ 0, 0 ]  sat=[ 0, 0 ]  lim="[-5 5  0 ]"  v0=[1.04 1.2612]
      settings: LibrarySourceBlock=sps_lib/Electrical Machines/Synchronous Machine Control/Excitation System
  Multi-Band Power System Stabilizer : spsMultiBandPowerSystemStabilizerLib/Multi-Band Power System Stabilizer  OperationMode=Simplified settings  Kg=k8  GL=[k9 k10]  GI=[k11 k12]  GH=[k13 k14]  GLd=[66 66 9.4]  TcLF=[1.667 2 0 0 0 0 2 2.4 0 0 0 0 1 1]  GId=[66 66 47.6]  TcIF=[1 1 0.25 0.3 0 0 1 1 0.3 0.36 0 0 0 0]  GHd=[66 66 233]  TcHF="[0.01 0.012 0 0 0 0  0.012 0.0144 0 0 0 0 1 1]"  LIM=[.075 .15 .15 .15]  Plot_On=off  MagdB_On=off  FreqRange=logspace(-2,2,500)
      settings: LibrarySourceBlock=|
      | sps_lib/Electrical Machines/Synchronous Machine Control/Multi-Band
      | Power System Stabilizer
  Multiport Switch1 : MultiPortSwitch  Inputs=2  SaturateOnIntegerOverflow=off
  PSS model3 : Constant  Value=0
  PSS model4 : Constant
  Real-Imag to Complex : RealImagToComplex
  STG1 : spsSteamTurbineandGovernorLib/Steam Turbine and Governor  gentype=Tandem-compound (single mass)  reg1="[ 1  0.05    0 ]"  reg2="[ 0.001  0.15 ]"  reg3="[ -0.1  0.1  0  4.496 ]"  N=3600  turb1="[ 0  10   3.3   0.5   ]"  turb2="[   0   0.36    0.36   0.28   ]"  HA="[ 0.046  1.430  1.465   0.192 ]"  KA="[ 90.44  53.88  64.59   62.94  ]"  DA="[ 0.0115  0.3575  0.3663   0.0137  ]"  ini1=0.52238  ini2=[0.779316,-31.4247]
      settings: LibrarySourceBlock=|
      | sps_lib/Electrical Machines/Synchronous Machine Control/Steam Turbine
      | and Governor
  Sum2 : Sum  InputSameDT=on  SaturateOnIntegerOverflow=on  OutDataTypeStr=Inherit: Same as first input
  Terminator : Terminator
  Terminator1 : Terminator
  Terminator2 : Terminator
  wref : Constant
  Pm1 : Outport  InitialOutput=0
  Vf1 : Outport  Port=2  InitialOutput=0
  tag scope: EFD1=global, Pe1=global, Q1=global, Vt1=global, d_theta1=global, pss1=global, theta1=global, w1=global
  wires:
  Bus Selector/7 -> EXCITATION1/3, Real-Imag to Complex/2  "<Stator voltage  vq (pu)>"
  wref/1 -> STG1/1
  Pref1/1 -> STG1/2
  m/1 -> Bus Selector/1
  Vref1/1 -> EXCITATION1/1
  EXCITATION1/1 -> Vf1/1, [EFD1]
  Real-Imag to Complex/1 -> [Vt1]
  Bus Selector/5 -> [theta1]  "<Rotor mechanical angle  theta (deg)>"
  Bus Selector/6 -> Real-Imag to Complex/1, EXCITATION1/2  "<Stator voltage  vd (pu)>"
  STG1/3 -> Terminator/1
  STG1/4 -> Pm1/1
  STG1/2 -> Terminator1/1
  STG1/1 -> Terminator2/1
  Bus Selector/1 -> [w1], STG1/3  "<Rotor speed  wm  (pu)>"
  Bus Selector/2 -> [d_theta1], STG1/4  "<Rotor angle deviation  d_theta (rad)>"
  Bus Selector/3 -> [Pe1]  "<Electrical power  Pe (pu)>"
  Bus Selector/8 -> [Q1]  "<Output reactive power  Qeo (pu)>"
  PSS1/1 -> Sum2/1
  Sum2/1 -> Multiport Switch1/1
  PSS model4/1 -> Sum2/2
  Multi-Band Power System Stabilizer/1 -> Multiport Switch1/3
  PSS model3/1 -> Multiport Switch1/2
  Multiport Switch1/1 -> [pss1], EXCITATION1/4
  Bus Selector/4 -> Multi-Band Power System Stabilizer/1  "<Rotor speed deviation  dw (pu)>"

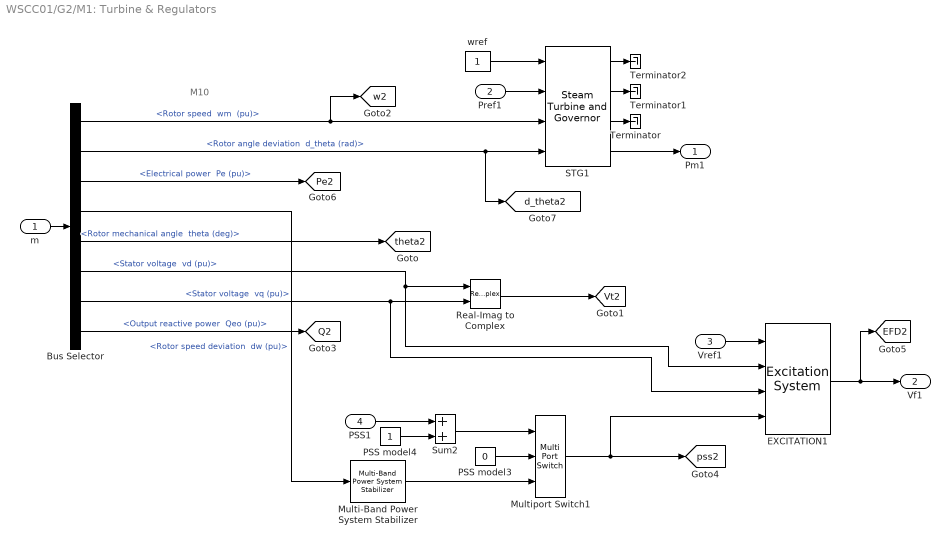
== system WSCC01/G2/M1: Turbine & Regulators ==
  note: M10
  m : Inport
  Pref1 : Inport  Port=2
  Vref1 : Inport  Port=3
  PSS1 : Inport  Port=4
  Bus Selector : BusSelector  OutputSignals="Mechanical.Rotor speed  wm  (pu),Mechanical.Rotor angle deviation  d_theta (rad),Mechanical.Electrical power  Pe (pu),Mechanical.Rotor speed deviation  dw (pu),Mechanical.Rotor mechanical angle  theta (deg),dq0 components.Stator voltage  vd (pu),dq0 components.Stator voltage  vq (pu),Output reactive power  Qeo (pu)"
  EXCITATION1 : spsExcitationSystemLib/Excitation System  tr=0.01  reg=[ 20 .2 ]  exc=[ 1, 0.314 ]  tgr="[10    1]"  damp=[ 0.63, 0.35 ]  sat=[ 0, 0 ]  lim=[ -5 5 0 ]  v0=[1.025 1.0912]
      settings: LibrarySourceBlock=sps_lib/Electrical Machines/Synchronous Machine Control/Excitation System
  Multi-Band Power System Stabilizer : spsMultiBandPowerSystemStabilizerLib/Multi-Band Power System Stabilizer  OperationMode=Simplified settings  Kg=k15  GL=[k16 k17]  GI=[k18 k19]  GH=[k20 k21]  GLd=[66 66 9.4]  TcLF=[1.667 2 0 0 0 0 2 2.4 0 0 0 0 1 1]  GId=[66 66 47.6]  TcIF=[1 1 0.25 0.3 0 0 1 1 0.3 0.36 0 0 0 0]  GHd=[66 66 233]  TcHF="[0.01 0.012 0 0 0 0  0.012 0.0144 0 0 0 0 1 1]"  LIM=[.075 .15 .15 .15]  Plot_On=off  MagdB_On=off  FreqRange=logspace(-2,2,500)
      settings: LibrarySourceBlock=|
      | sps_lib/Electrical Machines/Synchronous Machine Control/Multi-Band
      | Power System Stabilizer
  Multiport Switch1 : MultiPortSwitch  Inputs=2  SaturateOnIntegerOverflow=off
  PSS model3 : Constant  Value=0
  PSS model4 : Constant
  Real-Imag to Complex : RealImagToComplex
  STG1 : spsSteamTurbineandGovernorLib/Steam Turbine and Governor  gentype=Tandem-compound (single mass)  reg1="[ 1  0.05    0 ]"  reg2="[ 0.001  0.15 ]"  reg3="[ -0.1  0.1  0  4.496 ]"  N=3600  turb1="[ 0  10   3.3   0.5   ]"  turb2="[   0   0.36    0.36   0.28   ]"  HA="[ 0.046  1.430  1.465   0.192 ]"  KA="[ 90.44  53.88  64.59   62.94  ]"  DA="[ 0.0115  0.3575  0.3663   0.0137  ]"  ini1=0.52334  ini2=[0.779316,-31.4247]
      settings: LibrarySourceBlock=|
      | sps_lib/Electrical Machines/Synchronous Machine Control/Steam Turbine
      | and Governor
  Sum2 : Sum  InputSameDT=on  SaturateOnIntegerOverflow=on  OutDataTypeStr=Inherit: Same as first input
  Terminator : Terminator
  Terminator1 : Terminator
  Terminator2 : Terminator
  wref : Constant
  Pm1 : Outport  InitialOutput=0
  Vf1 : Outport  Port=2  InitialOutput=0
  tag scope: EFD2=global, Pe2=global, Q2=global, Vt2=global, d_theta2=global, pss2=global, theta2=global, w2=global
  wires:
  Bus Selector/7 -> EXCITATION1/3, Real-Imag to Complex/2  "<Stator voltage  vq (pu)>"
  wref/1 -> STG1/1
  Pref1/1 -> STG1/2
  m/1 -> Bus Selector/1
  Vref1/1 -> EXCITATION1/1
  EXCITATION1/1 -> Vf1/1, [EFD2]
  Real-Imag to Complex/1 -> [Vt2]
  Bus Selector/5 -> [theta2]  "<Rotor mechanical angle  theta (deg)>"
  Bus Selector/6 -> Real-Imag to Complex/1, EXCITATION1/2  "<Stator voltage  vd (pu)>"
  STG1/3 -> Terminator/1
  STG1/4 -> Pm1/1
  STG1/2 -> Terminator1/1
  STG1/1 -> Terminator2/1
  Bus Selector/1 -> [w2], STG1/3  "<Rotor speed  wm  (pu)>"
  Bus Selector/2 -> [d_theta2], STG1/4  "<Rotor angle deviation  d_theta (rad)>"
  Bus Selector/3 -> [Pe2]  "<Electrical power  Pe (pu)>"
  Bus Selector/8 -> [Q2]  "<Output reactive power  Qeo (pu)>"
  PSS1/1 -> Sum2/1
  Sum2/1 -> Multiport Switch1/1
  PSS model4/1 -> Sum2/2
  Multi-Band Power System Stabilizer/1 -> Multiport Switch1/3
  PSS model3/1 -> Multiport Switch1/2
  Multiport Switch1/1 -> [pss2], EXCITATION1/4
  Bus Selector/4 -> Multi-Band Power System Stabilizer/1  "<Rotor speed deviation  dw (pu)>"

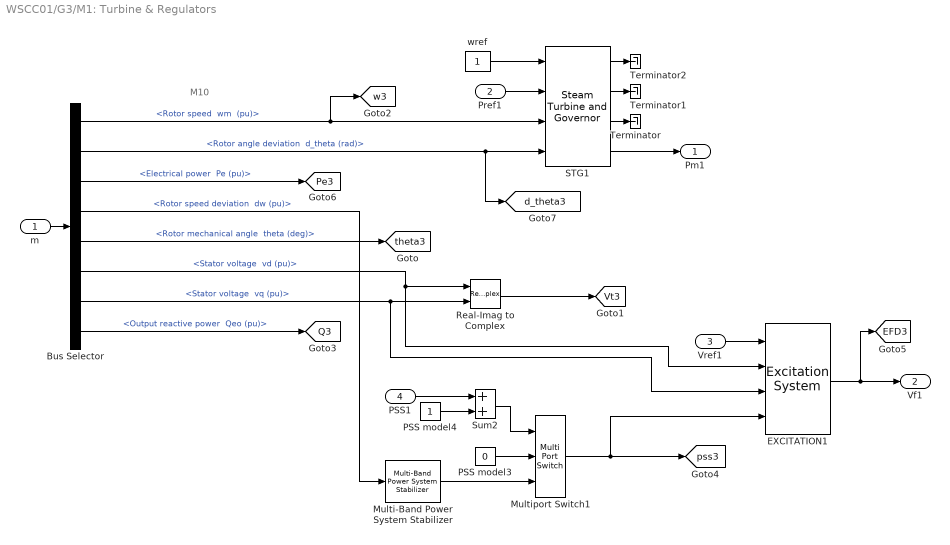
== system WSCC01/G3/M1: Turbine & Regulators ==
  note: M10
  m : Inport
  Pref1 : Inport  Port=2
  Vref1 : Inport  Port=3
  PSS1 : Inport  Port=4
  Bus Selector : BusSelector  OutputSignals="Mechanical.Rotor speed  wm  (pu),Mechanical.Rotor angle deviation  d_theta (rad),Mechanical.Electrical power  Pe (pu),Mechanical.Rotor speed deviation  dw (pu),Mechanical.Rotor mechanical angle  theta (deg),dq0 components.Stator voltage  vd (pu),dq0 components.Stator voltage  vq (pu),Output reactive power  Qeo (pu)"
  EXCITATION1 : spsExcitationSystemLib/Excitation System  tr=0.01  reg=[20 .2]  exc=[ 1, 0.314 ]  tgr=[ 10 1]  damp=[ 0.063, 0.35 ]  sat=[ 0, 0 ]  lim="[ -5 5  0 ]"  v0=[1.025 1.2407]
      settings: LibrarySourceBlock=sps_lib/Electrical Machines/Synchronous Machine Control/Excitation System
  Multi-Band Power System Stabilizer : spsMultiBandPowerSystemStabilizerLib/Multi-Band Power System Stabilizer  OperationMode=Simplified settings  Kg=k1  GL=[k2 k3]  GI=[k4 k5]  GH=[k6 k7]  GLd=[66 66 9.4]  TcLF=[1.667 2 0 0 0 0 2 2.4 0 0 0 0 1 1]  GId=[66 66 47.6]  TcIF=[1 1 0.25 0.3 0 0 1 1 0.3 0.36 0 0 0 0]  GHd=[66 66 233]  TcHF="[0.01 0.012 0 0 0 0  0.012 0.0144 0 0 0 0 1 1]"  LIM=[.075 .15 .15 .15]  Plot_On=off  MagdB_On=off  FreqRange=logspace(-2,2,500)
      settings: LibrarySourceBlock=|
      | sps_lib/Electrical Machines/Synchronous Machine Control/Multi-Band
      | Power System Stabilizer
  Multiport Switch1 : MultiPortSwitch  Inputs=2  SaturateOnIntegerOverflow=off
  PSS model3 : Constant  Value=0
  PSS model4 : Constant
  Real-Imag to Complex : RealImagToComplex
  STG1 : spsSteamTurbineandGovernorLib/Steam Turbine and Governor  gentype=Tandem-compound (single mass)  reg1="[ 1  0.05    0 ]"  reg2="[ 0.001  0.15 ]"  reg3="[ -0.1  0.1  0  4.496 ]"  N=3600  turb1="[ 0  10   3.3   0.5   ]"  turb2="[   0   0.36    0.36   0.28   ]"  HA="[ 0.046  1.430  1.465   0.192 ]"  KA="[ 90.44  53.88  64.59   62.94  ]"  DA="[ 0.0115  0.3575  0.3663   0.0137  ]"  ini1=0.69623  ini2=[0.779316,-31.4247]
      settings: LibrarySourceBlock=|
      | sps_lib/Electrical Machines/Synchronous Machine Control/Steam Turbine
      | and Governor
  Sum2 : Sum  InputSameDT=on  SaturateOnIntegerOverflow=on  OutDataTypeStr=Inherit: Same as first input
  Terminator : Terminator
  Terminator1 : Terminator
  Terminator2 : Terminator
  wref : Constant
  Pm1 : Outport  InitialOutput=0
  Vf1 : Outport  Port=2  InitialOutput=0
  tag scope: EFD3=global, Pe3=global, Q3=global, Vt3=global, d_theta3=global, pss3=global, theta3=global, w3=global
  wires:
  Bus Selector/4 -> Multi-Band Power System Stabilizer/1  "<Rotor speed deviation  dw (pu)>"
  Multiport Switch1/1 -> EXCITATION1/4, [pss3]
  PSS model3/1 -> Multiport Switch1/2
  Multi-Band Power System Stabilizer/1 -> Multiport Switch1/3
  PSS model4/1 -> Sum2/2
  Sum2/1 -> Multiport Switch1/1
  PSS1/1 -> Sum2/1
  Bus Selector/8 -> [Q3]  "<Output reactive power  Qeo (pu)>"
  Bus Selector/3 -> [Pe3]  "<Electrical power  Pe (pu)>"
  Bus Selector/2 -> STG1/4, [d_theta3]  "<Rotor angle deviation  d_theta (rad)>"
  Bus Selector/1 -> STG1/3, [w3]  "<Rotor speed  wm  (pu)>"
  STG1/1 -> Terminator2/1
  STG1/2 -> Terminator1/1
  STG1/4 -> Pm1/1
  STG1/3 -> Terminator/1
  Bus Selector/6 -> EXCITATION1/2, Real-Imag to Complex/1  "<Stator voltage  vd (pu)>"
  Bus Selector/5 -> [theta3]  "<Rotor mechanical angle  theta (deg)>"
  Real-Imag to Complex/1 -> [Vt3]
  EXCITATION1/1 -> [EFD3], Vf1/1
  Vref1/1 -> EXCITATION1/1
  m/1 -> Bus Selector/1
  Pref1/1 -> STG1/2
  wref/1 -> STG1/1
  Bus Selector/7 -> Real-Imag to Complex/2, EXCITATION1/3  "<Stator voltage  vq (pu)>"
